simulink model "Heartbridge"  (R2024b)
settings: Solver=ode45  StartTime=0.0  StopTime=1.68  MaxStep=0.5*Ts  RelTol=1e-3
values from neighbouring files (symbols this model uses):
  accel_limit = 16.5/L_ball    (= 1299.21259843)    [simulinkSetup.m]
  b = 286.8    [simulinkSetup.m]
  eta_ball = 0.8    [simulinkSetup.m]
  g = -9.81    [simulinkSetup.m]
  iLimit = 1.2*tau_max_ball    (= 1.75965508886)    [simulinkSetup.m]
  iRateLimit = -1    [simulinkSetup.m]
  J_eff_ball = J_m + J_ball + m_ball*p_ball^2/eta_ball    (= 1.28745416186e-05)    [simulinkSetup.m]
  k = 10490    [simulinkSetup.m]
  K_torque = (3/2)*(1/sqrt(3))*(60/(2*pi))/K_v    [simulinkSetup.m]
  L_ball = 12.7*1e-3    (= 0.0127)    [simulinkSetup.m]
  m_ball = 2    [simulinkSetup.m]
  p_ball = L_ball/(2*pi)    (= 0.00202126777727)    [simulinkSetup.m]
  pid_dq_hz = 100    [simulinkSetup.m]
  pid_kd = 0.05    [simulinkSetup.m]
  pid_ki = 0    [simulinkSetup.m]
  pid_kp = 6    [simulinkSetup.m]
  R_phase = 0.047    [simulinkSetup.m]
  servo_max_current = 40    [simulinkSetup.m]
  tau_d = 1.5*Ts    (= 0.0001)    [simulinkSetup.m]
  tau_max_ball = (F_max + m_ball*g)*p_ball/eta_ball    (= 1.46637924071)    [simulinkSetup.m]
  Ts = 1/servo_pwm_rate_hz    (= 6.66666666667e-05)    [simulinkSetup.m]
  V_batt = 18    [simulinkSetup.m]
  vel_limit = 0.6/L_ball    (= 47.2440944882)    [simulinkSetup.m]
  w_n_pll = 2*pi*f_pll/2.48    (= 1013.41698503)    [simulinkSetup.m]
  zeta_pll = 1    [simulinkSetup.m]
undefined symbols (not defined in the file or in its folder): DiscIntNeverNeededParam
libraries: simulink x6
settings Model: Creator=danie  LastModifiedBy=danie

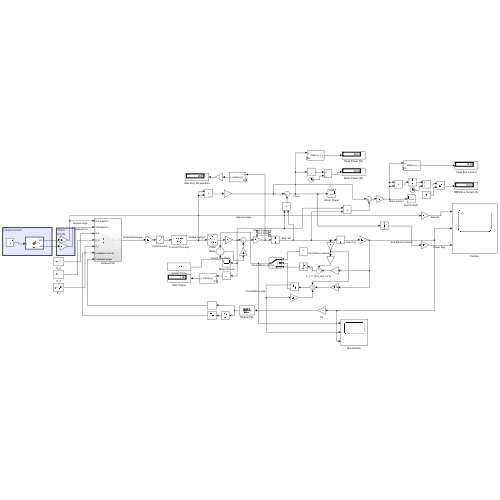
[thumbnail: Simulink's stored preview of the top-level diagram]
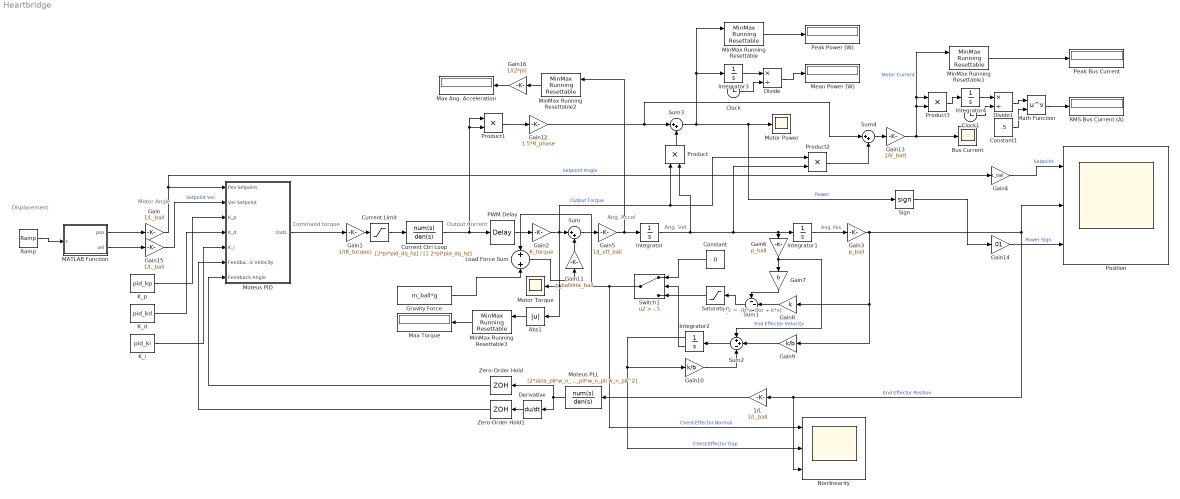
== system Heartbridge ==
  note: F_c = -(b*x_dot + k*x)
  note: Ang. Vel
  note: Ang. Accel
  note: Output Current
  note: Command torque
  note: Motor
      | Angle
  note: Displacement
  1/L : Gain  Gain=1/L_ball
  Abs1 : Abs  SaturateOnIntegerOverflow=off
  Bus Current : Scope
  Clock : Clock
  Clock1 : Clock
  Constant : Constant  Value=0
  Constant1 : Constant  Value=.5
  Current Ctrl Loop : TransferFcn  Numerator=[2*pi*pid_dq_hz]  Denominator=[1 2*pi*pid_dq_hz]
  Current Limit : Saturate  UpperLimit=servo_max_current  LowerLimit=-servo_max_current
  Derivative : Derivative
  Divide : Product  Inputs=*/
  Divide1 : Product  Inputs=*/
  Gain : Gain  Gain=1/L_ball
  Gain1 : Gain  Gain=1/(K_torque)
  Gain10 : Gain  Gain=k/b
  Gain11 : Gain  Gain=p_ball/eta_ball
  Gain12 : Gain  Gain=1.5*R_phase
  Gain13 : Gain  Gain=1/V_batt
  Gain14 : Gain  Gain=.01
  Gain15 : Gain  Gain=1/L_ball
  Gain16 : Gain  Gain=1/(2*pi)
  Gain2 : Gain  Gain=K_torque
  Gain3 : Gain  Gain=p_ball
  Gain4 : Gain  Gain=L_ball
  Gain5 : Gain  Gain=1/J_eff_ball
  Gain6 : Gain  Gain=p_ball
  Gain7 : Gain  Gain=b
  Gain8 : Gain  Gain=k
  Gain9 : Gain  Gain=k/b
  Gravity Force : Constant  Value=m_ball*g
  Integrator{,1,3..4} (4 alike) : Integrator
  Integrator2 : Integrator  LimitOutput=on  LowerSaturationLimit=0  ShowSaturationPort=on
  K_d : Constant  Value=pid_kd
  K_i : Constant  Value=pid_ki
  K_p : Constant  Value=pid_kp
  Load Force Sum : Sum
  MATLAB Function : MATLAB Function  TreatAsAtomicUnit=on
  Math Function : Math  Operator=pow
  Max Ang. Acceleration : Display
  Max Torque : Display
  Mean Power (W) : Display
  MinMax Running Resettable{,1..3} (4 alike) : simulink/Math Operations/MinMax Running Resettable  Function=max  vinit=0.0
  Moteus PID : Subsystem
  Moteus PLL : TransferFcn  Numerator=[2*zeta_pll*w_n_pll w_n_pll^2]  Denominator=[1 2*zeta_pll*w_n_pll w_n_pll^2]
  Motor Power : Scope
  Motor Torque : Scope
  Nonlinearity : Scope  NumInputPorts=3
  PWM Delay : TransportDelay  DelayTime=tau_d
  Peak Bus Current : Display
  Peak Power (W) : Display
  Position : Scope  NumInputPorts=3
  Product{,1..3} (4 alike) : Product
  RMS Bus Current (A) : Display
  Ramp : simulink/Sources/Ramp  slope=1  start=0  InitialOutput=0
  Saturation : Saturate  UpperLimit=inf  LowerLimit=0
  Sign : Signum
  Sum : Sum  Inputs=|++
  Sum1 : Sum  Inputs=--|
  Sum2 : Sum  Inputs=++-
  Sum3 : Sum  Inputs=|++
  Sum4 : Sum  Inputs=|++
  Switch1 : Switch  Criteria=u2 > Threshold  Threshold=-.5  SaturateOnIntegerOverflow=off  InputSameDT=off
  Zero-Order Hold : ZeroOrderHold  SampleTime=Ts
  Zero-Order Hold1 : ZeroOrderHold  SampleTime=Ts
  wires:
  Ramp/1 -> MATLAB Function/1(t)
  MATLAB Function/1(pos) -> Gain/1
  Gain/1 -> Moteus PID/1(Pos Setpoint), Gain4/1  "Setpoint Angle"
  K_p/1 -> Moteus PID/3(K_p)
  K_d/1 -> Moteus PID/4(K_d)
  K_i/1 -> Moteus PID/5(K_i)
  Moteus PID/1(Out1) -> Gain1/1
  Gain1/1 -> Current Limit/1
  Current Limit/1 -> Current Ctrl Loop/1
  Current Ctrl Loop/1 -> Product1/2, Product1/1, PWM Delay/1
  PWM Delay/1 -> Gain2/1
  Moteus PLL/1 -> Zero-Order Hold/1, Derivative/1
  Derivative/1 -> Zero-Order Hold1/1
  Zero-Order Hold1/1 -> Moteus PID/6(Feedback Velocity)
  Zero-Order Hold/1 -> Moteus PID/7(Feedback Angle)
  Gain3/1 -> Gain9/1, Gain8/1, Nonlinearity/3, 1/L/1, Position/2  "End Effector Position"
  1/L/1 -> Moteus PLL/1
  Gain4/1 -> Position/1  "Setpoint"
  Gain2/1 -> Abs1/1, Motor Torque/1, Product/1, Product2/1, Sum/1  "Output Torque"
  Sum/1 -> Gain5/1
  Integrator/1 -> Product/2, Integrator1/1, Gain6/1, Product2/2
  Integrator1/1 -> Gain3/1  "Ang. Pos"
  Gain6/1 -> Sum2/1, Gain7/1  "End Effector Velocity"
  Gain7/1 -> Sum1/1
  Gain8/1 -> Sum1/2
  Sum1/1 -> Saturation/1
  Gain9/1 -> Sum2/2
  Sum2/1 -> Integrator2/1
  Integrator2/2 -> Switch1/2
  Saturation/1 -> Switch1/3
  Constant/1 -> Switch1/1
  Gain10/1 -> Sum2/3
  Integrator2/1 -> Nonlinearity/2, Gain10/1  "Chest-Effector Gap"
  Gain11/1 -> Sum/2
  Switch1/1 -> Nonlinearity/1, Load Force Sum/1  "Chest-Effector Normal"
  Product/1 -> Sum3/2
  Product1/1 -> Gain12/1
  Gain12/1 -> Sum4/1, Sum3/1
  Sum3/1 -> Sign/1, Motor Power/1, Integrator3/1, MinMax Running Resettable/1  "Power"
  Divide/1 -> Mean Power (W)/1
  MinMax Running Resettable/1 -> Peak Power (W)/1
  Product2/1 -> Sum4/2
  Sum4/1 -> Gain13/1
  Gain13/1 -> MinMax Running Resettable1/1, Product3/1, Product3/2, Bus Current/1  "Motor Current"
  Math Function/1 -> RMS Bus Current (A)/1
  Integrator3/1 -> Divide/1
  Clock/1 -> Divide/2
  Product3/1 -> Integrator4/1
  Integrator4/1 -> Divide1/1
  Clock1/1 -> Divide1/2
  Divide1/1 -> Math Function/1
  Constant1/1 -> Math Function/2
  MinMax Running Resettable1/1 -> Peak Bus Current/1
  Gain5/1 -> MinMax Running Resettable2/1, Integrator/1
  MinMax Running Resettable2/1 -> Gain16/1
  MATLAB Function/2(vel) -> Gain15/1
  MinMax Running Resettable3/1 -> Max Torque/1
  Abs1/1 -> MinMax Running Resettable3/1
  Sign/1 -> Gain14/1
  Gain14/1 -> Position/3  "Power Sign"
  Gain15/1 -> Moteus PID/2(Vel Setpoint)  "Setpoint Vel"
  Gain16/1 -> Max Ang. Acceleration/1
  Gravity Force/1 -> Load Force Sum/2
  Load Force Sum/1 -> Gain11/1

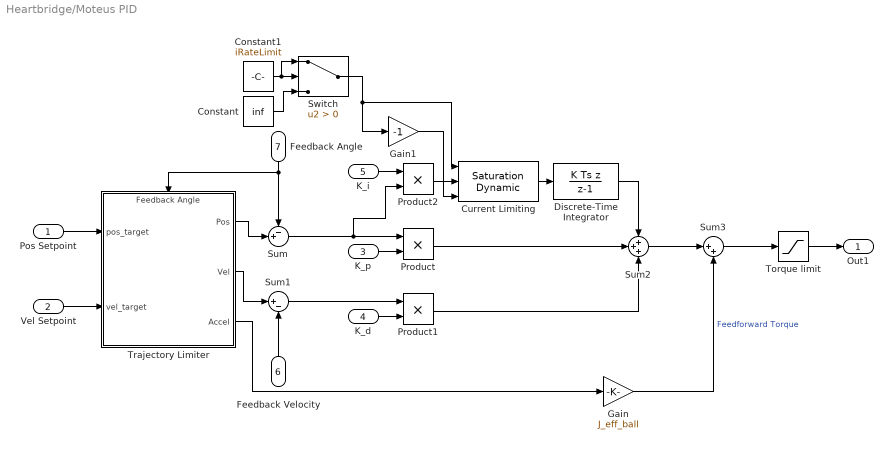
== system Heartbridge/Moteus PID ==
  Pos Setpoint : Inport
  Vel Setpoint : Inport  Port=2
  K_p : Inport  Port=3
  K_d : Inport  Port=4
  K_i : Inport  Port=5
  Feedback Velocity : Inport  Port=6
  Feedback Angle : Inport  Port=7
  Constant : Constant  Value=inf
  Constant1 : Constant  Value=iRateLimit
  Current Limiting : simulink/Discontinuities/Saturation Dynamic  OutMin=[]  OutMax=[]  OutDataTypeStr=Inherit: Same as second input  OutDataType=fixdt(1, 16)  OutScaling=2^-10  DoSatur=off
  Discrete-Time Integrator : DiscreteIntegrator  IntegratorMethod=Integration: Backward Euler  SampleTime=-1  LimitOutput=on  UpperSaturationLimit=iLimit  LowerSaturationLimit=-iLimit  ICPrevOutput=DiscIntNeverNeededParam  ICPrevScaledInput=DiscIntNeverNeededParam
  Gain : Gain  Gain=J_eff_ball
  Gain1 : Gain  Gain=-1
  Product : Product
  Product1 : Product
  Product2 : Product
  Sum : Sum  Inputs=-+|
  Sum1 : Sum  Inputs=|+-
  Sum2 : Sum  Inputs=+++
  Sum3 : Sum  Inputs=|++
  Switch : Switch  Criteria=u2 > Threshold  SaturateOnIntegerOverflow=off  InputSameDT=off
  Torque limit : Saturate  UpperLimit=tau_max_ball  LowerLimit=-tau_max_ball
  Trajectory Limiter : Subsystem
      settings: PortSchema="{\"entries\":[{\"content\":{\"sides\":[{\"content\":{\"connectorIds\":[\"In1\",\"In2\"]},\"type\":\"ConnectorPlacement.EquallySpacedRectSide\",\"uuid\":\"61548264-7453-4a29-bd66-f960738fac7f\"},{\"content\":{\"connectorIds\":[\"Out1\",\"Out2\",\"Out3\"],\"side\":\"RIGHT\"},\"type\":\"ConnectorPlacement.EquallySpacedRectSide\",\"uuid\":\"f716a689-e738-4715-bb87-0b02ddc273b1\"},{\"content\":{\"connectorIds\":[\"In3\"],\"side\":\"TOP\"},\"type\":\"ConnectorPlacement.EquallySpacedRectSide\",\"uuid\":\"a8aad9a9-d98c-4bd5-94ec-230b36f09c6d\"}]},\"type\":\"ConnectorPlacement.EquallySpacedConnector\",\"uuid\":\"a20a297a-1ecc-4216-a539-303763b08d57\"}],\"packageUris\":[\"http://schema.mathworks.com/mf0/Connector/R2020b\"],\"version\":\"1.0\"}"
  Out1 : Outport
  wires:
  Feedback Angle/1 -> Trajectory Limiter/3(Feedback Angle), Sum/1
  Feedback Velocity/1 -> Sum1/2
  K_p/1 -> Product/2
  K_d/1 -> Product1/2
  Sum1/1 -> Product1/1
  Sum/1 -> Product2/2, Product/1
  Product/1 -> Sum2/2
  Product1/1 -> Sum2/3
  Constant1/1 -> Switch/1, Switch/2
  Constant/1 -> Switch/3
  Switch/1 -> Gain1/1, Current Limiting/1
  Gain1/1 -> Current Limiting/3
  Sum2/1 -> Sum3/1
  Gain/1 -> Sum3/2  "Feedforward Torque"
  Sum3/1 -> Torque limit/1
  Torque limit/1 -> Out1/1
  K_i/1 -> Product2/1
  Product2/1 -> Current Limiting/2
  Current Limiting/1 -> Discrete-Time Integrator/1
  Discrete-Time Integrator/1 -> Sum2/1
  Pos Setpoint/1 -> Trajectory Limiter/1(pos_target)
  Trajectory Limiter/1(Pos) -> Sum/2
  Trajectory Limiter/2(Vel) -> Sum1/1
  Vel Setpoint/1 -> Trajectory Limiter/2(vel_target)
  Trajectory Limiter/3(Accel) -> Gain/1

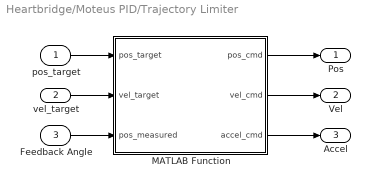
== system Heartbridge/Moteus PID/Trajectory Limiter ==
  pos_target : Inport
  vel_target : Inport  Port=2
  Feedback Angle : Inport  Port=3
  MATLAB Function : MATLAB Function  TreatAsAtomicUnit=on
  Pos : Outport
  Vel : Outport  Port=2
  Accel : Outport  Port=3
  wires:
  MATLAB Function/3(accel_cmd) -> Accel/1
  MATLAB Function/2(vel_cmd) -> Vel/1
  MATLAB Function/1(pos_cmd) -> Pos/1
  pos_target/1 -> MATLAB Function/1(pos_target)
  Feedback Angle/1 -> MATLAB Function/3(pos_measured)
  vel_target/1 -> MATLAB Function/2(vel_target)

== matlab function Heartbridge/Moteus PID/Trajectory Limiter/MATLAB Function ==
  settings: updateMethod=DISCRETE  sampleTime=Ts
  data: pos_target input; vel_target input; pos_cmd output; pos_measured input; vel_cmd output; accel_cmd output; Ts parameter; vel_limit parameter; accel_limit parameter
function [pos_cmd, vel_cmd, accel_cmd] = moteus_trajectory_limiter( ...
        pos_target, vel_target, pos_measured, Ts, vel_limit, accel_limit)
% moteus trajectory limiter (fw/bldc_servo_position.h: UpdateCommand /
% UpdateTrajectory / DoVelocityAndAccelLimits)
% Negative or NaN limits mean "disabled", as in the firmware.
%   pos_target  : commanded position [rev]
%   vel_target  : commanded velocity sent with the position [rev/s]
%   pos_measured: measured position, used only on the first call [rev]
% Planning is done in the target's frame (the target moves at vel_target).
% Assumes the command is re-sent every Ts, so pos_target already advances.

  persistent pos_state vel_state is_done last_target last_vel
  accel_on = isfinite(accel_limit) && accel_limit >= 0;
  vel_on   = isfinite(vel_limit)   && vel_limit   >= 0;

  % ---- Both limits off: pass the command straight through ----
  if ~accel_on && ~vel_on
    pos_state = pos_target;  vel_state = vel_target;
    pos_cmd = pos_target;  vel_cmd = vel_target;  accel_cmd = 0;
    return;
  end

  if isempty(pos_state)
    pos_state = pos_measured;  vel_state = 0;
    is_done = false;  last_target = pos_target;  last_vel = vel_target;
  end
  % A new command restarts the trajectory
  if pos_target ~= last_target || vel_target ~= last_vel
    is_done = false;  last_target = pos_target;  last_vel = vel_target;
  end

  % Clamp the target velocity to the velocity limit
  vf = vel_target;
  if vel_on, vf = min(max(vf, -vel_limit), vel_limit); end

  % ---- Trajectory complete: continue at the target velocity ----
  if is_done
    pos_state = pos_state + vel_state * Ts;
    pos_cmd = pos_state;  vel_cmd = vel_state;  accel_cmd = 0;
    return;
  end

  dx = pos_target - pos_state;
  v0 = vel_state;

  % ---- Velocity limit only: move at constant +/- vel_limit ----
  if ~accel_on
    s0 = 1 - 2*(dx < 0);                      % +1 if dx >= 0, else -1
    vel_state = s0 * vel_limit;
    if (1 - 2*((dx - vel_state*Ts) < 0)) ~= s0  % this step reaches the target
      vel_state = vf;  is_done = true;
    end
    pos_state = pos_state + vel_state * Ts;
    pos_cmd = pos_state;  vel_cmd = vel_state;  accel_cmd = 0;
    return;
  end

  % ---- Acceleration limit (velocity limit inf if unset) ----
  a = accel_limit;
  if vel_on, vlim = vel_limit; else, vlim = inf; end

  v_frame = v0 - vf;                  % velocity relative to the target
  cs = 1 - 2*(v_frame >= 0);          % copysign(1, -v_frame)
  if abs(v0) > vlim
    accel = -sign(v0) * a;            % overspeed: slow to the limit first
  elseif v_frame * dx >= 0 && dx ~= 0
    % Moving towards the target (in the target frame)
    stop_distance = v_frame^2 / (2 * a);
    req_decel     = v_frame^2 / (2 * abs(dx));
    if abs(dx) > stop_distance
      v_next   = abs(v_frame) + a * Ts;
      dx_after = abs(dx) - (abs(v_frame) + v_next) / 2 * Ts;
      if dx_after < v_next^2 / (2 * a)
        accel = cs * min(a, req_decel);   % switch to braking this step
      elseif abs(v0) < vlim
        accel = sign(dx) * a;
      else
        accel = 0;                        % at velocity limit: cruise
      end
    else
      accel = cs * min(a, req_decel);
    end
  else
    accel = cs * a;                   % moving away: fix that
  end

  vel_state = v0 + accel * Ts;
  v1 = vel_state;
  % Spend at least one step exactly at the velocity limit
  if vel_on && min(abs(v0), abs(v1)) < vlim && max(abs(v0), abs(v1)) > vlim
    vel_state = sign(v1) * vlim;  accel = 0;
  end

  % Done once velocity reaches the target velocity near the target
  target_cross  = min(v0, vel_state) <= vf && max(v0, vel_state) >= vf;
  target_near   = abs(vel_state - vf) < a * 0.5 * Ts;
  position_near = abs(dx) <= max(abs(vel_state - vf), abs(vf)) * 10 * Ts;
  if (target_cross || target_near) && position_near
    vel_state = vf;  accel = 0;  is_done = true;
  end

  if accel ~= 0
    pos_state = pos_state + (v0 + vel_state) / 2 * Ts;
  else
    pos_state = pos_state + vel_state * Ts;
  end

  pos_cmd = pos_state;  vel_cmd = vel_state;  accel_cmd = accel;
end

== matlab function Heartbridge/MATLAB Function ==
  data: t input; pos output; vel output
function [pos, vel] = fcn(t)
    time = mod(t, .56);
    
    if (time <= .12)
        pos = 0;
        vel = 0;
    elseif (time <= .24)
        pos = (-41.6666667*(time - .12))*1e-2;
        vel = -41.6666667e-2;
    elseif (time <= .323)
        pos = -5e-2;
        vel = 0;
    else
        pos = (21.0965609*(time - .323) - 5)*1e-2;
        vel = 21.0965609e-2;
    end
end
